simulink model "ejemplo_lotka_volterra"  (R2025a)
settings: Solver=VariableStepAuto  StartTime=0.0  StopTime=400  RelTol=1e-3
settings Model: Creator=cmparedesv  LastModifiedBy=cmparedesv

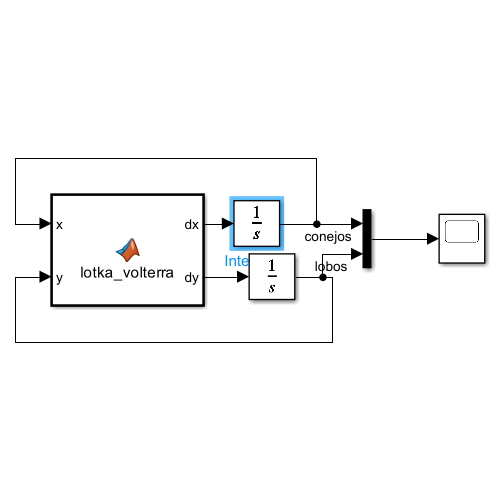
[thumbnail: Simulink's stored preview of the top-level diagram]
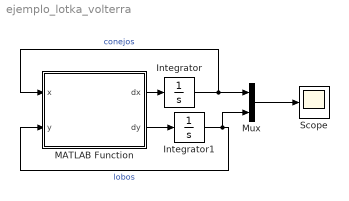
== system ejemplo_lotka_volterra ==
  Integrator : Integrator  InitialCondition=10
  Integrator1 : Integrator  InitialCondition=2
  MATLAB Function : MATLAB Function  TreatAsAtomicUnit=on
  Mux : Mux  Inputs=2
  Scope : Scope
      settings: ActiveDisplayYMinimum=-1.6916448213663688  ActiveDisplayYMaximum=15.227702178659165
  wires:
  MATLAB Function/1(dx) -> Integrator/1
  Integrator/1 -> Mux/1, MATLAB Function/1(x)  "conejos"
  MATLAB Function/2(dy) -> Integrator1/1
  Integrator1/1 -> Mux/2, MATLAB Function/2(y)  "lobos"
  Mux/1 -> Scope/1

== matlab function ejemplo_lotka_volterra/MATLAB Function ==
  data: x input; dx output; y input; dy output
function [dx,dy] = lotka_volterra(x,y)
%parametros del sistema
a = 2;
b= 4;
c= 5;
d= 6;
dx = x*(a-b*y);
dy = -y*(c-d*x);
